simulink model "untitled"  (R2023b)
settings: Solver=VariableStepAuto  StartTime=0.0  StopTime=10.0  RelTol=1e-3
settings Model: Creator=hp  LastModifiedBy=hp

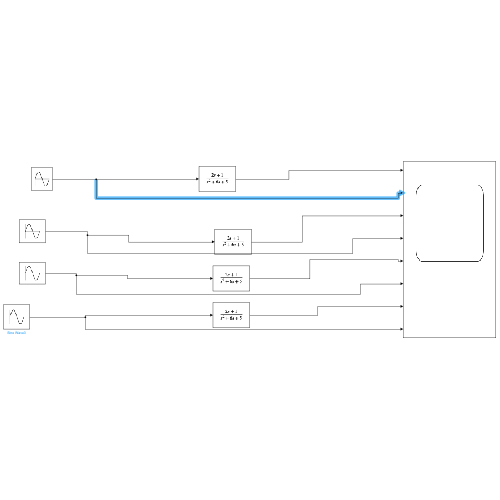
[thumbnail: Simulink's stored preview of the top-level diagram]
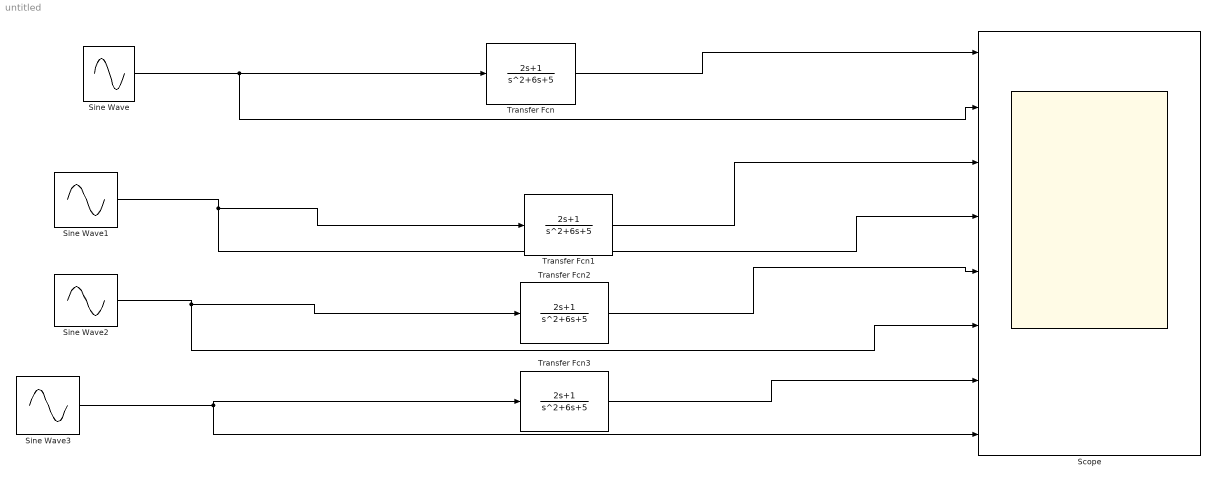
== system untitled ==
  Scope : Scope  NumInputPorts=8
  Sine Wave : Sin  SampleTime=0
  Sine Wave1 : Sin  Frequency=10  SampleTime=0
  Sine Wave2 : Sin  Frequency=100  SampleTime=0
  Sine Wave3 : Sin  Frequency=1000  SampleTime=0
  Transfer Fcn{,1..3} (4 alike) : TransferFcn  Numerator=[2 1]  Denominator=[1 6 5]
  wires:
  Transfer Fcn/1 -> Scope/1
  Sine Wave/1 -> Scope/2, Transfer Fcn/1
  Sine Wave3/1 -> Scope/8, Transfer Fcn3/1
  Transfer Fcn3/1 -> Scope/7
  Sine Wave1/1 -> Transfer Fcn1/1, Scope/4
  Sine Wave2/1 -> Transfer Fcn2/1, Scope/6
  Transfer Fcn1/1 -> Scope/3
  Transfer Fcn2/1 -> Scope/5
